simulink model "T2_Simulink"  (R2026a)
settings: Solver=VariableStepAuto  StopTime=2
settings Model: Creator=diyar  LastModifiedBy=diyar

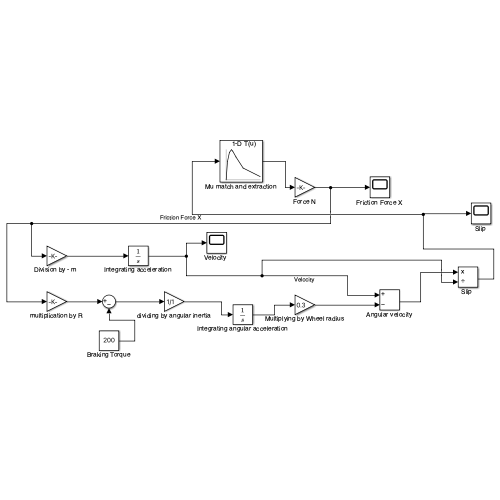
[thumbnail: Simulink's stored preview of the top-level diagram]
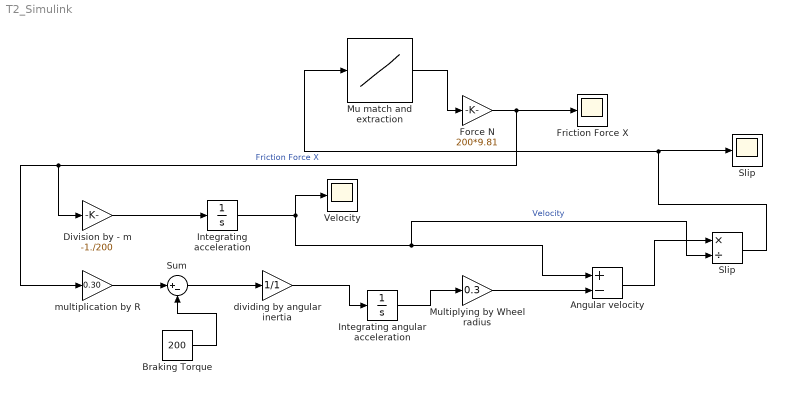
== system T2_Simulink ==
  Angular velocity : Sum  Inputs=+-
  Braking Torque : Constant  Value=200
  "Division by - m " : Gain  Gain=-1./200
  Force N : Gain  Gain=200*9.81
  Friction Force X : Scope
      settings: ActiveDisplayYMinimum=-78.810685112492422  ActiveDisplayYMaximum=709.29616601239854
  Integrating acceleration : Integrator  InitialCondition=25  UpperSaturationLimit=1  LowerSaturationLimit=0
  Integrating angular acceleration : Integrator  InitialCondition=25/0.3
  Mu match and extraction : Lookup_n-D  NumberOfTableDimensions=1  BreakpointsForDimension1=[0;0.050000000000000003;0.10000000000000001;0.14999999999999999;0.20000000000000001;0.29999999999999999;0.5;1]  Table=[0;0.59999999999999998;0.90000000000000002;1;0.94999999999999996;0.75;0.40000000000000002;0.10000000000000001]  InternalRulePriority=Speed  RndMeth=Simplest
  Multiplying by Wheel radius : Gain  Gain=0.3
  Slip : Scope
      settings: ActiveDisplayYMinimum=-0.0033473787424606028  ActiveDisplayYMaximum=0.030126408682144012
  "Slip " : Product  Inputs=*/
  Sum : Sum  Inputs=|+-
  "Velocity " : Scope
      settings: ActiveDisplayYMinimum=17.924062537263449  ActiveDisplayYMaximum=25.786215273637396  DataLoggingVariableName=ScopeData2
  dividing by angular inertia : Gain  Gain=1/1
  multiplication by R : Gain  Gain=0.30
  wires:
  Integrating acceleration/1 -> "Slip "/2, Angular velocity/1, "Velocity "/1  "Velocity"
  "Division by - m "/1 -> Integrating acceleration/1
  multiplication by R/1 -> Sum/1
  Force N/1 -> Friction Force X/1, multiplication by R/1, "Division by - m "/1  "Friction Force X"
  Braking Torque/1 -> Sum/2
  Sum/1 -> dividing by angular inertia/1
  dividing by angular inertia/1 -> Integrating angular acceleration/1
  Integrating angular acceleration/1 -> Multiplying by Wheel radius/1
  Multiplying by Wheel radius/1 -> Angular velocity/2
  Angular velocity/1 -> "Slip "/1
  Mu match and extraction/1 -> Force N/1
  "Slip "/1 -> Slip/1, Mu match and extraction/1
